simulink model "simulation"  (R2023a)
settings: Solver=FixedStepAuto  StartTime=0.0  StopTime=10.0  FixedStep=1e-3  RelTol=1e-3
PreLoadFcn:
  | init_pms;
InitFcn:
  | init_pms
settings Model: Creator=user  LastModifiedBy=user

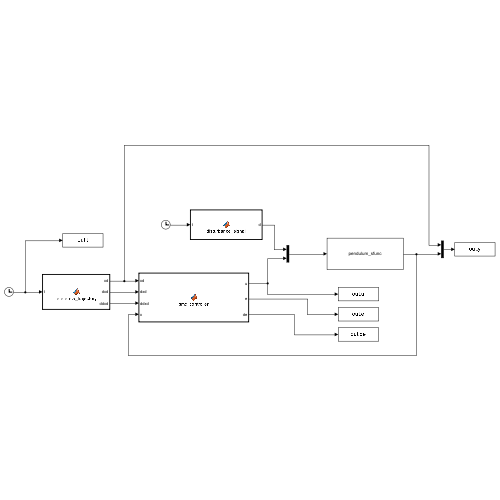
[thumbnail: Simulink's stored preview of the top-level diagram]
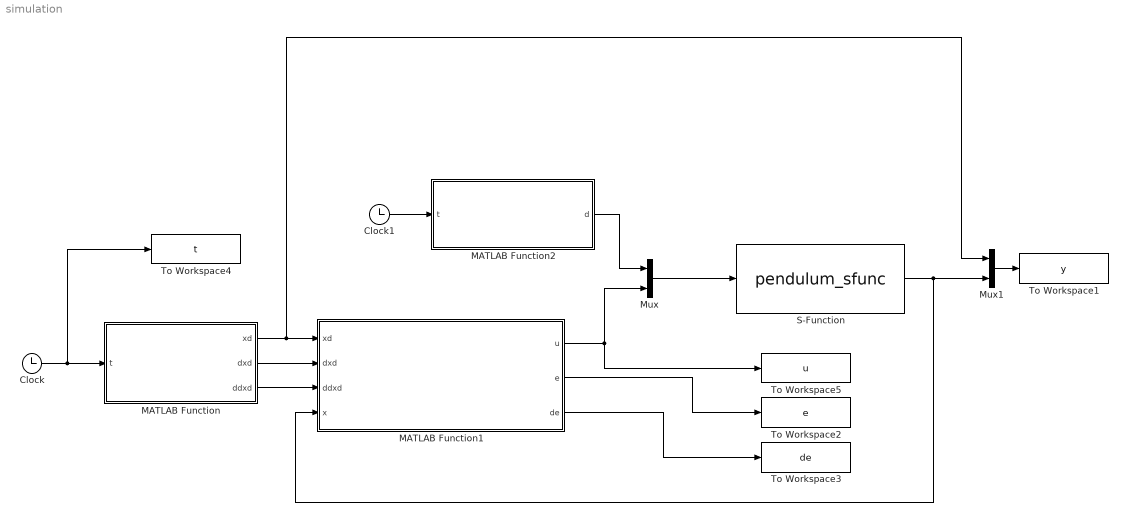
== system simulation ==
  Clock : Clock
  Clock1 : Clock
  MATLAB Function : MATLAB Function  TreatAsAtomicUnit=on
  MATLAB Function1 : MATLAB Function  TreatAsAtomicUnit=on
  MATLAB Function2 : MATLAB Function  TreatAsAtomicUnit=on
  Mux : Mux  Inputs=2
  Mux1 : Mux  Inputs=2
  S-Function : S-Function  FunctionName=pendulum_sfunc  Parameters=pms  SFunctionDeploymentMode=off  EnableBusSupport=off
  To Workspace1 : ToWorkspace  VariableName=y  SampleTime=-1
      settings: Save2DSignal=2-D array (concatenate along first dimension)
  To Workspace2 : ToWorkspace  VariableName=e  SampleTime=-1
      settings: Save2DSignal=2-D array (concatenate along first dimension)
  To Workspace3 : ToWorkspace  VariableName=de  SampleTime=-1
      settings: Save2DSignal=2-D array (concatenate along first dimension)
  To Workspace4 : ToWorkspace  VariableName=t  SampleTime=-1
      settings: Save2DSignal=2-D array (concatenate along first dimension)
  To Workspace5 : ToWorkspace  VariableName=u  SampleTime=-1
      settings: Save2DSignal=2-D array (concatenate along first dimension)
  wires:
  Clock/1 -> To Workspace4/1, MATLAB Function/1(t)
  MATLAB Function/1(xd) -> Mux1/1, MATLAB Function1/1(xd)
  MATLAB Function/2(dxd) -> MATLAB Function1/2(dxd)
  MATLAB Function/3(ddxd) -> MATLAB Function1/3(ddxd)
  Clock1/1 -> MATLAB Function2/1(t)
  MATLAB Function1/1(u) -> To Workspace5/1, Mux/2
  MATLAB Function2/1(d) -> Mux/1
  Mux/1 -> S-Function/1
  S-Function/1 -> Mux1/2, MATLAB Function1/4(x)
  Mux1/1 -> To Workspace1/1
  MATLAB Function1/2(e) -> To Workspace2/1
  MATLAB Function1/3(de) -> To Workspace3/1

== matlab function simulation/MATLAB Function1 ==
  data: xd input; dxd input; ddxd input; x input; u output; e output; de output; pms parameter
function [u, e, de] = smc_controller(xd, dxd, ddxd, x, pms)
[u, e, de] = smc_controller(x, xd, dxd, ddxd, pms);

== matlab function simulation/MATLAB Function ==
  data: t input; xd output; dxd output; ddxd output
function [xd, dxd, ddxd] = reference_trajectory(t)
[xd, dxd, ddxd] = reference_trajectory(t);

== matlab function simulation/MATLAB Function2 ==
  data: t input; d output
function d = disturbance_signal(t)
d = disturbance_signal(t);
